simulink model "mpc_ctrl"  (R2025b)
settings: Solver=FixedStepDiscrete  StartTime=0.0  StopTime=10.0  FixedStep=0.01  RelTol=1e-3
undefined symbols (not defined in the file or in its folder): mpc_motor_init
settings Model: Creator=jnune  LastModifiedBy=jnune
settings OptimizationCC: DefaultParameterBehavior=Inlined  EnhancedBackFolding=on  PassReuseOutputArgsAs=Individual arguments  ZeroExternalMemoryAtStartup=off  ZeroInternalMemoryAtStartup=off  MaxStackSize=64  OptimizeBlockOrder=speed  DifferentSizesBufferReuse=on  OptimizationCustomize=off  EfficientTunableParamExpr=on
settings DebuggingCC: ParameterPrecisionLossMsg=none  ParameterTunabilityLossMsg=error
settings HardwareCC: ProdBitPerPointer=32.0  ProdBitPerSizeT=32.0  ProdBitPerPtrDiffT=32.0  ProdLargestAtomicInteger=Long  ProdLargestAtomicFloat=Double  ProdWordSize=32.0  ProdLongLongMode=on  ProdHWDeviceType=ARM Compatible->ARM Cortex-M
settings ModelReferenceCC: ModelReferenceNumInstancesAllowed=Single  SupportModelReferenceSimTargetCustomCode=on
settings SFSimCC: SimCustomHeaderCode="#include \"mpc_motor.h\""  MATLABDynamicMemAlloc=off
settings SFSimCC: SimUserSources=|
  | C:\Escritorio\Memoria\MPC_OSQP_simple\mpc_motor.c
  | C:\Escritorio\Memoria\MPC_OSQP_simple\osqp\src\auxil.c
  | C:\Escritorio\Memoria\MPC_OSQP_simple\osqp\src\error.c
  | C:\Escritorio\Memoria\MPC_OSQP_simple\osqp\src\lin_alg.c
  | C:\Escritorio\Memoria\MPC_OSQP_simple\osqp\src\osqp.c
  | C:\Escritorio\Memoria\MPC_OSQP_simple\osqp\src\proj.c
  | C:\Escritorio\Memoria\MPC_OSQP_simple\osqp\src\qdldl.c
  | C:\Escritorio\Memoria\MPC_OSQP_simple\osqp\src\qdldl_interface.c
  | C:\Escritorio\Memoria\MPC_OSQP_simple\osqp\src\scaling.c
  | C:\Escritorio\Memoria\MPC_OSQP_simple\osqp\src\util.c
  | C:\Escritorio\Memoria\MPC_OSQP_simple\osqp\src\workspace.c
settings SFSimCC: SimUserIncludeDirs=|
  | C:\Escritorio\Memoria\MPC_OSQP_simple
  | C:\Escritorio\Memoria\MPC_OSQP_simple\osqp\include
settings RTWCC: SystemTargetFile=ert.tlc  HardwareBoard=STM32 Nucleo F767ZI  TemplateMakefile=ert_default_tmf  CustomHeaderCode="#include \"mpc_motor.h\""  Toolchain=GNU Tools for ARM Embedded Processors  Description=Embedded Coder
settings RTWCC: CustomInclude=|
  | C:\Escritorio\Memoria\MPC_OSQP_simple
  | C:\Escritorio\Memoria\MPC_OSQP_simple\osqp\include
settings RTWCC: CustomSource=|
  | C:\Escritorio\Memoria\MPC_OSQP_simple\mpc_motor.c
  | C:\Escritorio\Memoria\MPC_OSQP_simple\osqp\src\auxil.c
  | C:\Escritorio\Memoria\MPC_OSQP_simple\osqp\src\error.c
  | C:\Escritorio\Memoria\MPC_OSQP_simple\osqp\src\lin_alg.c
  | C:\Escritorio\Memoria\MPC_OSQP_simple\osqp\src\osqp.c
  | C:\Escritorio\Memoria\MPC_OSQP_simple\osqp\src\proj.c
  | C:\Escritorio\Memoria\MPC_OSQP_simple\osqp\src\qdldl.c
  | C:\Escritorio\Memoria\MPC_OSQP_simple\osqp\src\qdldl_interface.c
  | C:\Escritorio\Memoria\MPC_OSQP_simple\osqp\src\scaling.c
  | C:\Escritorio\Memoria\MPC_OSQP_simple\osqp\src\util.c
  | C:\Escritorio\Memoria\MPC_OSQP_simple\osqp\src\workspace.c
settings CodeAppCC: ForceParamTrailComments=on  IgnoreCustomStorageClasses=off  OperatorAnnotations=on  SimulinkDataObjDesc=on  SFDataObjDesc=on  InsertBlockDesc=on
settings ERTTargetCC: ExtModeTransport=3.0  ExtModeStaticAlloc=on  ExtModeStaticAllocSize=2000.0  ExtModeMexFile=ext_xcp  ExtModeIntrfLevel=Level2 - Open  TargetLangStandard=C99 (ISO)  SubcomponentCodeInterfacePackaging=Nonreusable function

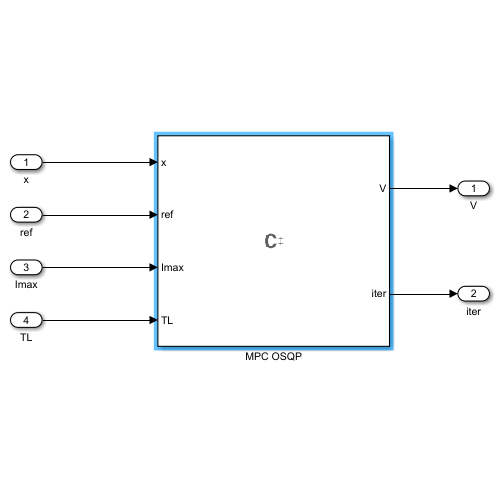
[thumbnail: Simulink's stored preview of the top-level diagram]
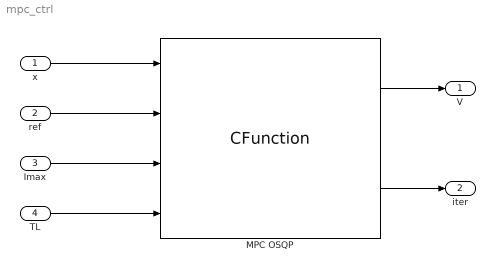
== system mpc_ctrl ==
  x : Inport  PortDimensions=2  SampleTime=0.01
  ref : Inport  Port=2  PortDimensions=1  SampleTime=0.01
  Imax : Inport  Port=3  PortDimensions=1  SampleTime=0.01
  TL : Inport  Port=4  PortDimensions=1  SampleTime=0.01
  MPC OSQP : CFunction  OutputCode=|  StartCode=mpc_motor_init();  CodegenOutputCode=|  CodegenStartCode=mpc_motor_init();  SampleTime=0.01  CustomCodeSettingLocation=ModelConfigurationParameters
      OutputCode=|
      | double v;
      | iter = mpc_motor_step(x, ref, Imax, TL, &v);
      | V = v;
      CodegenOutputCode=|
      | double v;
      | iter = mpc_motor_step(x, ref, Imax, TL, &v);
      | V = v;
  V : Outport
  iter : Outport  Port=2
  wires:
  x/1 -> MPC OSQP/1
  ref/1 -> MPC OSQP/2
  Imax/1 -> MPC OSQP/3
  TL/1 -> MPC OSQP/4
  MPC OSQP/1 -> V/1
  MPC OSQP/2 -> iter/1
